simulink model "projectile_frott"  (R2026a)
settings: Solver=FixedStepAuto  StartTime=0  StopTime=10  FixedStep=1/10
values from neighbouring files (symbols this model uses):
  coef_frot = 0.04    [parametres_TP_projectile.m]
  g = 9.81    [parametres_TP_projectile.m]
  M = 15    [parametres_TP_projectile.m]
  pos_x0 = 0    [Projectile_parameters.m]    (also in parametres_TP_projectile.m)
  pos_y0 = 0    [Projectile_parameters.m]    (also in parametres_TP_projectile.m)
  vit_x0 = vit0*cos(theta)    [Projectile_parameters.m]    (also in parametres_TP_projectile.m)
  vit_y0 = vit0*sin(theta)    [Projectile_parameters.m]    (also in parametres_TP_projectile.m)
settings Model: Creator=lulu1  LastModifiedBy=lulu1

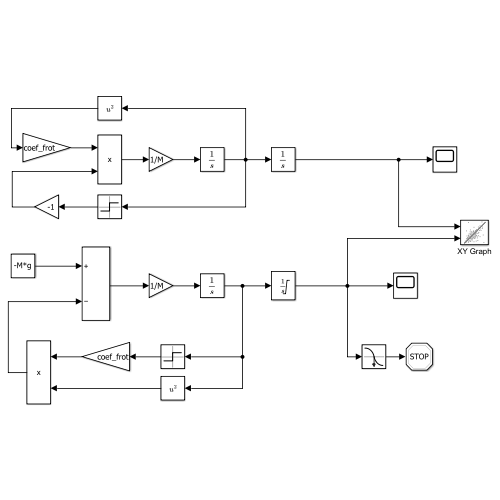
[thumbnail: Simulink's stored preview of the top-level diagram]
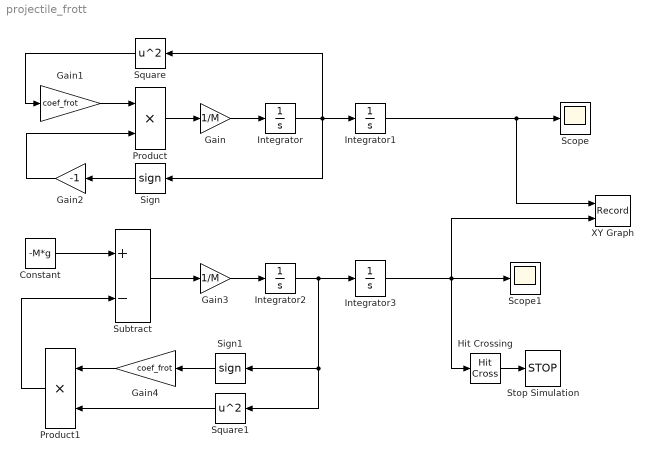
== system projectile_frott ==
  Constant : Constant  Value=-M*g
  Gain : Gain  Gain=1/M
  Gain1 : Gain  Gain=coef_frot
  Gain2 : Gain  Gain=-1
  Gain3 : Gain  Gain=1/M
  Gain4 : Gain  Gain=coef_frot
  Hit Crossing : HitCross  HitCrossingDirection=falling
  Integrator : Integrator  InitialCondition=vit_x0
  Integrator1 : Integrator  InitialCondition=pos_x0
  Integrator2 : Integrator  InitialCondition=vit_y0
  Integrator3 : Integrator  InitialCondition=pos_y0  LimitOutput=on  LowerSaturationLimit=0
  Product : Product
  Product1 : Product
  Scope : Scope
      settings: ActiveDisplayYMinimum=-1  ActiveDisplayYMaximum=1
  Scope1 : Scope
  Sign : Signum
  Sign1 : Signum
  Square : Math  Operator=square
  Square1 : Math  Operator=square
  Stop Simulation : Stop
  Subtract : Sum  Inputs=+-
  XY Graph : Record  NumPorts=2.0  FileSettingsInternal="{\"entries\":[{\"content\":{\"excelSettings\":{\"content\":{},\"type\":\"Streamout.ExcelSettings\"},\"parquetSettings\":{\"content\":{},\"type\":\"Streamout.ParquetSettings\"}},\"type\":\"Streamout.FileSettingStorage\",\"uuid\":\"\"}],\"packageUris\":[\"http:\\/\\/schema.mathworks.com\\/mf0\\/streamout_blocks\\/R2020a\"],\"version\":\"1.0\"}"  FrameSettings=[0, 0]  Layout=[1 1]  SignalsInternal="{\"entries\":[{\"content\":{\"signals\":[{\"content\":{\"blockPath\":[],\"dimensions\":[1],\"domain\":\"\",\"lineColor\":\"#a2142f\",\"plots\":[ 1 ],\"port\":1,\"sid\":[\"\"],\"signalID\":1,\"signalName\":\"Integrator1\"},\"type\":\"RecordBlkView.Signal\",\"uuid\":\"\"},{\"content\":{\"blockPath\":[],\"dimensions\":[1],\"domain\":\"\",\"lineColor\":\"#139fff\",\"plots\":[ 1 ],\"port\":2,\"sid\":[\"\"],\"signalID\":2,\"signalName\":\"Integrator3\"},\"type\":\"RecordBlkView.Signal\",\"uuid\":\"\"}]},\"type\":\"RecordBlkView.InputSignals\",\"uuid\":\"\"}],\"packageUris\":[\"http:\\/\\/schema.mathworks.com\\/mf0\\/streamout_blocks\\/R2020a\"],\"version\":\"1.0\"}"  VisualizationBindings="{\"xyplotplugin\":{\"info\":[{\"series\":[{\"bindingParametersList\":[{\"parameter\":\"X-Axis\",\"signalID\":1,\"signalName\":\"Integrator1\"},{\"parameter\":\"Y-Axis\",\"signalID\":2,\"signalName\":\"Integrator3\"}],\"seriesID\":0}],\"subplotID\":1}]}}"  CompatibilityTag=XY
  wires:
  Integrator/1 -> Square/1, Integrator1/1, Sign/1
  Gain/1 -> Integrator/1
  Product/1 -> Gain/1
  Gain1/1 -> Product/1
  Square/1 -> Gain1/1
  Sign/1 -> Gain2/1
  Gain2/1 -> Product/2
  Constant/1 -> Subtract/1
  Integrator2/1 -> Square1/1, Sign1/1, Integrator3/1
  Gain3/1 -> Integrator2/1
  Subtract/1 -> Gain3/1
  Product1/1 -> Subtract/2
  Gain4/1 -> Product1/1
  Sign1/1 -> Gain4/1
  Square1/1 -> Product1/2
  Integrator3/1 -> XY Graph/2, Scope1/1, Hit Crossing/1
  Integrator1/1 -> XY Graph/1, Scope/1
  Hit Crossing/1 -> Stop Simulation/1
